simulink model "afe_rst_inv_psm_distributed_control_two_delays"  (R2026a)
settings: Solver=ode1be  StopTime=simlength  FixedStep=tc  MaxStep=Tc
values from neighbouring files (symbols this model uses):
  Amplitude_U = 1.16    [grid_fault_generator.m]
  Amplitude_V = Amplitude_U    (= 1.16)    [grid_fault_generator.m]
  Amplitude_W = Amplitude_U    (= 1.16)    [grid_fault_generator.m]
  end_time_LVRT = start_time_LVRT + error_length    [grid_fault_generator.m]
  Igrid_phase_normalization_factor = 270*sqrt(2)    [grid_emulator.m]
  omega_grid_emulator_nom = w_grid    (= 314.159265359)    [grid_emulator.m]
  omega_grid_nom = w_grid    (= 314.159265359)    [grid_emulator.m]
  t_ramp = 20e-3    (= 0.02)    [grid_fault_generator.m]
  ugrid_factor = 1    [grid_emulator.m]
  V_phase_normalization_factor = Vgrid_phase_normalization_factor    [grid_emulator.m]
  Vdc_bez = 1070    [grid_emulator.m]
  Vemu_ref_norm = Vemu_ref * sqrt(2) / V_phase_normalization_factor    [grid_emulator.m]
  vn_eta_pu = 0    [grid_emulator.m]
  vn_xi_pu = 0    [grid_emulator.m]
  vp_xi_pu = 1    [grid_emulator.m]
undefined symbols (not defined in the file or in its folder): Adrso, Aresd, Bresd, CFi, CFu, Cresd, Crso, CTRPIFF_CLIP_RELEASE, dead_time_INV, emf_fb_p, emf_fb_p_ccaller_1, emf_fb_p_ccaller_2, emf_p, emf_p_ccaller_1, emf_p_ccaller_2, fPWM_INV, g0_161Hz, g0_500Hz, g1_161Hz, g1_500Hz, i_grid_neg_eta_lim, i_grid_neg_eta_red_lim, i_grid_neg_xi_lim, i_grid_neg_xi_red_lim, i_grid_pos_eta_lim, i_grid_pos_eta_red_lim, ibez, id_lim, ieta_neg_ref_lim, ieta_pos_ref_lim, iq_lim, ixi_pos_ref_lim, Jm_norm, k_frt_ref, kg, ki_afe, ki_i, ki_id, ki_iq, ki_rc_neg_grid, ki_rc_pos_grid, ki_vs, ki_w, kp_afe, kp_i, kp_id, kp_iq, kp_rc_neg_grid, kp_rc_pos_grid, kp_vs, kp_w, kw, l1, l2, Lalpha_norm, Ld_norm, Ldrso, Lq_norm, Ls_norm, luenberger_l1 ... (+30)
libraries: fl_lib x146, nesl_utility x62, simulink x8, cstblocks_lti x7, sl_discontinuities x3, single_phase_transformer_lib x3, flexshaft_lib x1, permanent_magnet_synchronous_machine x1
(part 4 of 14)

== system afe_rst_inv_psm_distributed_control_two_delays/grid/instantaneus_power/moving_avarage1 ==
  In : Inport
  Gain1 : Gain  Gain=omega_grid_emulator_nom/2/pi  SaturateOnIntegerOverflow=on  OutDataTypeStr=Inherit: Same as input  ParamDataTypeStr=Inherit: Same as input
  Sum4 : Sum  SaturateOnIntegerOverflow=on
  Sum8 : Sum  Inputs=+-  InputSameDT=on  SaturateOnIntegerOverflow=on  OutDataTypeStr=Inherit: Same as first input
  Transport Delay : TransportDelay  DelayTime=2*pi/omega_grid_emulator_nom  BufferSize=2048*4  PadeOrder=2
  Unit Delay2 : UnitDelay  SampleTime=ts_afe
  kp2 : Gain  Gain=ts_afe  SaturateOnIntegerOverflow=on  OutDataTypeStr=Inherit: Same as input  ParamDataTypeStr=Inherit: Same as input
  Mean : Outport  VectorParamsAs1DForOutWhenUnconnected=off
  wires:
  Gain1/1 -> Mean/1
  kp2/1 -> Sum4/1
  Unit Delay2/1 -> Sum4/2
  In/1 -> kp2/1
  Sum8/1 -> Gain1/1
  Sum4/1 -> Unit Delay2/1, Transport Delay/1, Sum8/1
  Transport Delay/1 -> Sum8/2

== system afe_rst_inv_psm_distributed_control_two_delays/grid/instantaneus_power/rms ==
  In1 : Inport
  Gain : Gain  Gain=n10-1
  Gain1 : Gain  Gain=1/n10
  Math Function : Math  Operator=magnitude^2  SignedPower=on
  Sqrt : Sqrt
  Sum : Sum  Inputs=|++
  Unit Delay : UnitDelay  SampleTime=ts_afe
  Out1 : Outport  VectorParamsAs1DForOutWhenUnconnected=off
  wires:
  In1/1 -> Math Function/1
  Sum/1 -> Gain1/1
  Gain1/1 -> Sqrt/1, Unit Delay/1
  Unit Delay/1 -> Gain/1
  Math Function/1 -> Sum/1
  Sqrt/1 -> Out1/1
  Gain/1 -> Sum/2

== system afe_rst_inv_psm_distributed_control_two_delays/grid/instantaneus_power/rms1 ==
  In1 : Inport
  Gain : Gain  Gain=n10-1
  Gain1 : Gain  Gain=1/n10
  Math Function : Math  Operator=magnitude^2  SignedPower=on
  Sqrt : Sqrt
  Sum : Sum  Inputs=|++
  Unit Delay : UnitDelay  SampleTime=ts_afe
  Out1 : Outport  VectorParamsAs1DForOutWhenUnconnected=off
  wires:
  Gain/1 -> Sum/2
  Sqrt/1 -> Out1/1
  Math Function/1 -> Sum/1
  Unit Delay/1 -> Gain/1
  Gain1/1 -> Unit Delay/1, Sqrt/1
  Sum/1 -> Gain1/1
  In1/1 -> Math Function/1

== system afe_rst_inv_psm_distributed_control_two_delays/grid/instantaneus_power/rms2 ==
  In1 : Inport
  Gain : Gain  Gain=n10-1
  Gain1 : Gain  Gain=1/n10
  Math Function : Math  Operator=magnitude^2  SignedPower=on
  Sqrt : Sqrt
  Sum : Sum  Inputs=|++
  Unit Delay : UnitDelay  SampleTime=ts_afe
  Out1 : Outport  VectorParamsAs1DForOutWhenUnconnected=off
  wires:
  In1/1 -> Math Function/1
  Sum/1 -> Gain1/1
  Gain1/1 -> Sqrt/1, Unit Delay/1
  Unit Delay/1 -> Gain/1
  Math Function/1 -> Sum/1
  Sqrt/1 -> Out1/1
  Gain/1 -> Sum/2

== system afe_rst_inv_psm_distributed_control_two_delays/grid/instantaneus_power/rms3 ==
  In1 : Inport
  Gain : Gain  Gain=n10-1
  Gain1 : Gain  Gain=1/n10
  Math Function : Math  Operator=magnitude^2  SignedPower=on
  Sqrt : Sqrt
  Sum : Sum  Inputs=|++
  Unit Delay : UnitDelay  SampleTime=ts_afe
  Out1 : Outport  VectorParamsAs1DForOutWhenUnconnected=off
  wires:
  Gain/1 -> Sum/2
  Sqrt/1 -> Out1/1
  Math Function/1 -> Sum/1
  Unit Delay/1 -> Gain/1
  Gain1/1 -> Unit Delay/1, Sqrt/1
  Sum/1 -> Gain1/1
  In1/1 -> Math Function/1

== system afe_rst_inv_psm_distributed_control_two_delays/grid/instantaneus_power/rms4 ==
  In1 : Inport
  Gain : Gain  Gain=n10-1
  Gain1 : Gain  Gain=1/n10
  Math Function : Math  Operator=magnitude^2  SignedPower=on
  Sqrt : Sqrt
  Sum : Sum  Inputs=|++
  Unit Delay : UnitDelay  SampleTime=ts_afe
  Out1 : Outport  VectorParamsAs1DForOutWhenUnconnected=off
  wires:
  In1/1 -> Math Function/1
  Sum/1 -> Gain1/1
  Gain1/1 -> Sqrt/1, Unit Delay/1
  Unit Delay/1 -> Gain/1
  Math Function/1 -> Sum/1
  Sqrt/1 -> Out1/1
  Gain/1 -> Sum/2

== system afe_rst_inv_psm_distributed_control_two_delays/grid/instantaneus_power/rms5 ==
  In1 : Inport
  Gain : Gain  Gain=n10-1
  Gain1 : Gain  Gain=1/n10
  Math Function : Math  Operator=magnitude^2  SignedPower=on
  Sqrt : Sqrt
  Sum : Sum  Inputs=|++
  Unit Delay : UnitDelay  SampleTime=ts_afe
  Out1 : Outport  VectorParamsAs1DForOutWhenUnconnected=off
  wires:
  Gain/1 -> Sum/2
  Sqrt/1 -> Out1/1
  Math Function/1 -> Sum/1
  Unit Delay/1 -> Gain/1
  Gain1/1 -> Unit Delay/1, Sqrt/1
  Sum/1 -> Gain1/1
  In1/1 -> Math Function/1

== system afe_rst_inv_psm_distributed_control_two_delays/grid/sequences accordind to VDE411/moving_avarage ==
  In : Inport
  Gain1 : Gain  Gain=omega_grid_emulator_nom/2/pi  SaturateOnIntegerOverflow=on  OutDataTypeStr=Inherit: Same as input  ParamDataTypeStr=Inherit: Same as input
  Sum4 : Sum  SaturateOnIntegerOverflow=on
  Sum8 : Sum  Inputs=+-  InputSameDT=on  SaturateOnIntegerOverflow=on  OutDataTypeStr=Inherit: Same as first input
  Transport Delay : TransportDelay  DelayTime=2*pi/omega_grid_emulator_nom  BufferSize=2048*4  PadeOrder=2
  Unit Delay2 : UnitDelay  SampleTime=ts_afe
  kp2 : Gain  Gain=ts_afe  SaturateOnIntegerOverflow=on  OutDataTypeStr=Inherit: Same as input  ParamDataTypeStr=Inherit: Same as input
  Mean : Outport  VectorParamsAs1DForOutWhenUnconnected=off
  wires:
  Transport Delay/1 -> Sum8/2
  Sum4/1 -> Sum8/1, Transport Delay/1, Unit Delay2/1
  Sum8/1 -> Gain1/1
  In/1 -> kp2/1
  Unit Delay2/1 -> Sum4/2
  kp2/1 -> Sum4/1
  Gain1/1 -> Mean/1

== system afe_rst_inv_psm_distributed_control_two_delays/grid/sequences accordind to VDE411/moving_avarage1 ==
  In : Inport
  Gain1 : Gain  Gain=omega_grid_emulator_nom/2/pi  SaturateOnIntegerOverflow=on  OutDataTypeStr=Inherit: Same as input  ParamDataTypeStr=Inherit: Same as input
  Sum4 : Sum  SaturateOnIntegerOverflow=on
  Sum8 : Sum  Inputs=+-  InputSameDT=on  SaturateOnIntegerOverflow=on  OutDataTypeStr=Inherit: Same as first input
  Transport Delay : TransportDelay  DelayTime=2*pi/omega_grid_emulator_nom  BufferSize=2048*4  PadeOrder=2
  Unit Delay2 : UnitDelay  SampleTime=ts_afe
  kp2 : Gain  Gain=ts_afe  SaturateOnIntegerOverflow=on  OutDataTypeStr=Inherit: Same as input  ParamDataTypeStr=Inherit: Same as input
  Mean : Outport  VectorParamsAs1DForOutWhenUnconnected=off
  wires:
  Gain1/1 -> Mean/1
  kp2/1 -> Sum4/1
  Unit Delay2/1 -> Sum4/2
  In/1 -> kp2/1
  Sum8/1 -> Gain1/1
  Sum4/1 -> Unit Delay2/1, Transport Delay/1, Sum8/1
  Transport Delay/1 -> Sum8/2

== system afe_rst_inv_psm_distributed_control_two_delays/grid/sequences accordind to VDE411/moving_avarage10 ==
  In : Inport
  Gain1 : Gain  Gain=omega_grid_emulator_nom/2/pi  SaturateOnIntegerOverflow=on  OutDataTypeStr=Inherit: Same as input  ParamDataTypeStr=Inherit: Same as input
  Sum4 : Sum  SaturateOnIntegerOverflow=on
  Sum8 : Sum  Inputs=+-  InputSameDT=on  SaturateOnIntegerOverflow=on  OutDataTypeStr=Inherit: Same as first input
  Transport Delay : TransportDelay  DelayTime=2*pi/omega_grid_emulator_nom  BufferSize=2048*4  PadeOrder=2
  Unit Delay2 : UnitDelay  SampleTime=ts_afe
  kp2 : Gain  Gain=ts_afe  SaturateOnIntegerOverflow=on  OutDataTypeStr=Inherit: Same as input  ParamDataTypeStr=Inherit: Same as input
  Mean : Outport  VectorParamsAs1DForOutWhenUnconnected=off
  wires:
  Transport Delay/1 -> Sum8/2
  Sum4/1 -> Sum8/1, Transport Delay/1, Unit Delay2/1
  Sum8/1 -> Gain1/1
  In/1 -> kp2/1
  Unit Delay2/1 -> Sum4/2
  kp2/1 -> Sum4/1
  Gain1/1 -> Mean/1

== system afe_rst_inv_psm_distributed_control_two_delays/grid/sequences accordind to VDE411/moving_avarage11 ==
  In : Inport
  Gain1 : Gain  Gain=omega_grid_emulator_nom/2/pi  SaturateOnIntegerOverflow=on  OutDataTypeStr=Inherit: Same as input  ParamDataTypeStr=Inherit: Same as input
  Sum4 : Sum  SaturateOnIntegerOverflow=on
  Sum8 : Sum  Inputs=+-  InputSameDT=on  SaturateOnIntegerOverflow=on  OutDataTypeStr=Inherit: Same as first input
  Transport Delay : TransportDelay  DelayTime=2*pi/omega_grid_emulator_nom  BufferSize=2048*4  PadeOrder=2
  Unit Delay2 : UnitDelay  SampleTime=ts_afe
  kp2 : Gain  Gain=ts_afe  SaturateOnIntegerOverflow=on  OutDataTypeStr=Inherit: Same as input  ParamDataTypeStr=Inherit: Same as input
  Mean : Outport  VectorParamsAs1DForOutWhenUnconnected=off
  wires:
  Gain1/1 -> Mean/1
  kp2/1 -> Sum4/1
  Unit Delay2/1 -> Sum4/2
  In/1 -> kp2/1
  Sum8/1 -> Gain1/1
  Sum4/1 -> Unit Delay2/1, Transport Delay/1, Sum8/1
  Transport Delay/1 -> Sum8/2

== system afe_rst_inv_psm_distributed_control_two_delays/grid/sequences accordind to VDE411/moving_avarage2 ==
  In : Inport
  Gain1 : Gain  Gain=omega_grid_emulator_nom/2/pi  SaturateOnIntegerOverflow=on  OutDataTypeStr=Inherit: Same as input  ParamDataTypeStr=Inherit: Same as input
  Sum4 : Sum  SaturateOnIntegerOverflow=on
  Sum8 : Sum  Inputs=+-  InputSameDT=on  SaturateOnIntegerOverflow=on  OutDataTypeStr=Inherit: Same as first input
  Transport Delay : TransportDelay  DelayTime=2*pi/omega_grid_emulator_nom  BufferSize=2048*4  PadeOrder=2
  Unit Delay2 : UnitDelay  SampleTime=ts_afe
  kp2 : Gain  Gain=ts_afe  SaturateOnIntegerOverflow=on  OutDataTypeStr=Inherit: Same as input  ParamDataTypeStr=Inherit: Same as input
  Mean : Outport  VectorParamsAs1DForOutWhenUnconnected=off
  wires:
  Transport Delay/1 -> Sum8/2
  Sum4/1 -> Sum8/1, Transport Delay/1, Unit Delay2/1
  Sum8/1 -> Gain1/1
  In/1 -> kp2/1
  Unit Delay2/1 -> Sum4/2
  kp2/1 -> Sum4/1
  Gain1/1 -> Mean/1

== system afe_rst_inv_psm_distributed_control_two_delays/grid/sequences accordind to VDE411/moving_avarage3 ==
  In : Inport
  Gain1 : Gain  Gain=omega_grid_emulator_nom/2/pi  SaturateOnIntegerOverflow=on  OutDataTypeStr=Inherit: Same as input  ParamDataTypeStr=Inherit: Same as input
  Sum4 : Sum  SaturateOnIntegerOverflow=on
  Sum8 : Sum  Inputs=+-  InputSameDT=on  SaturateOnIntegerOverflow=on  OutDataTypeStr=Inherit: Same as first input
  Transport Delay : TransportDelay  DelayTime=2*pi/omega_grid_emulator_nom  BufferSize=2048*4  PadeOrder=2
  Unit Delay2 : UnitDelay  SampleTime=ts_afe
  kp2 : Gain  Gain=ts_afe  SaturateOnIntegerOverflow=on  OutDataTypeStr=Inherit: Same as input  ParamDataTypeStr=Inherit: Same as input
  Mean : Outport  VectorParamsAs1DForOutWhenUnconnected=off
  wires:
  Gain1/1 -> Mean/1
  kp2/1 -> Sum4/1
  Unit Delay2/1 -> Sum4/2
  In/1 -> kp2/1
  Sum8/1 -> Gain1/1
  Sum4/1 -> Unit Delay2/1, Transport Delay/1, Sum8/1
  Transport Delay/1 -> Sum8/2

== system afe_rst_inv_psm_distributed_control_two_delays/grid/sequences accordind to VDE411/moving_avarage4 ==
  In : Inport
  Gain1 : Gain  Gain=omega_grid_emulator_nom/2/pi  SaturateOnIntegerOverflow=on  OutDataTypeStr=Inherit: Same as input  ParamDataTypeStr=Inherit: Same as input
  Sum4 : Sum  SaturateOnIntegerOverflow=on
  Sum8 : Sum  Inputs=+-  InputSameDT=on  SaturateOnIntegerOverflow=on  OutDataTypeStr=Inherit: Same as first input
  Transport Delay : TransportDelay  DelayTime=2*pi/omega_grid_emulator_nom  BufferSize=2048*4  PadeOrder=2
  Unit Delay2 : UnitDelay  SampleTime=ts_afe
  kp2 : Gain  Gain=ts_afe  SaturateOnIntegerOverflow=on  OutDataTypeStr=Inherit: Same as input  ParamDataTypeStr=Inherit: Same as input
  Mean : Outport  VectorParamsAs1DForOutWhenUnconnected=off
  wires:
  Transport Delay/1 -> Sum8/2
  Sum4/1 -> Sum8/1, Transport Delay/1, Unit Delay2/1
  Sum8/1 -> Gain1/1
  In/1 -> kp2/1
  Unit Delay2/1 -> Sum4/2
  kp2/1 -> Sum4/1
  Gain1/1 -> Mean/1

== system afe_rst_inv_psm_distributed_control_two_delays/grid/sequences accordind to VDE411/moving_avarage5 ==
  In : Inport
  Gain1 : Gain  Gain=omega_grid_emulator_nom/2/pi  SaturateOnIntegerOverflow=on  OutDataTypeStr=Inherit: Same as input  ParamDataTypeStr=Inherit: Same as input
  Sum4 : Sum  SaturateOnIntegerOverflow=on
  Sum8 : Sum  Inputs=+-  InputSameDT=on  SaturateOnIntegerOverflow=on  OutDataTypeStr=Inherit: Same as first input
  Transport Delay : TransportDelay  DelayTime=2*pi/omega_grid_emulator_nom  BufferSize=2048*4  PadeOrder=2
  Unit Delay2 : UnitDelay  SampleTime=ts_afe
  kp2 : Gain  Gain=ts_afe  SaturateOnIntegerOverflow=on  OutDataTypeStr=Inherit: Same as input  ParamDataTypeStr=Inherit: Same as input
  Mean : Outport  VectorParamsAs1DForOutWhenUnconnected=off
  wires:
  Gain1/1 -> Mean/1
  kp2/1 -> Sum4/1
  Unit Delay2/1 -> Sum4/2
  In/1 -> kp2/1
  Sum8/1 -> Gain1/1
  Sum4/1 -> Unit Delay2/1, Transport Delay/1, Sum8/1
  Transport Delay/1 -> Sum8/2

== system afe_rst_inv_psm_distributed_control_two_delays/grid/sequences accordind to VDE411/moving_avarage6 ==
  In : Inport
  Gain1 : Gain  Gain=omega_grid_emulator_nom/2/pi  SaturateOnIntegerOverflow=on  OutDataTypeStr=Inherit: Same as input  ParamDataTypeStr=Inherit: Same as input
  Sum4 : Sum  SaturateOnIntegerOverflow=on
  Sum8 : Sum  Inputs=+-  InputSameDT=on  SaturateOnIntegerOverflow=on  OutDataTypeStr=Inherit: Same as first input
  Transport Delay : TransportDelay  DelayTime=2*pi/omega_grid_emulator_nom  BufferSize=2048*4  PadeOrder=2
  Unit Delay2 : UnitDelay  SampleTime=ts_afe
  kp2 : Gain  Gain=ts_afe  SaturateOnIntegerOverflow=on  OutDataTypeStr=Inherit: Same as input  ParamDataTypeStr=Inherit: Same as input
  Mean : Outport  VectorParamsAs1DForOutWhenUnconnected=off
  wires:
  Transport Delay/1 -> Sum8/2
  Sum4/1 -> Sum8/1, Transport Delay/1, Unit Delay2/1
  Sum8/1 -> Gain1/1
  In/1 -> kp2/1
  Unit Delay2/1 -> Sum4/2
  kp2/1 -> Sum4/1
  Gain1/1 -> Mean/1

== system afe_rst_inv_psm_distributed_control_two_delays/grid/sequences accordind to VDE411/moving_avarage7 ==
  In : Inport
  Gain1 : Gain  Gain=omega_grid_emulator_nom/2/pi  SaturateOnIntegerOverflow=on  OutDataTypeStr=Inherit: Same as input  ParamDataTypeStr=Inherit: Same as input
  Sum4 : Sum  SaturateOnIntegerOverflow=on
  Sum8 : Sum  Inputs=+-  InputSameDT=on  SaturateOnIntegerOverflow=on  OutDataTypeStr=Inherit: Same as first input
  Transport Delay : TransportDelay  DelayTime=2*pi/omega_grid_emulator_nom  BufferSize=2048*4  PadeOrder=2
  Unit Delay2 : UnitDelay  SampleTime=ts_afe
  kp2 : Gain  Gain=ts_afe  SaturateOnIntegerOverflow=on  OutDataTypeStr=Inherit: Same as input  ParamDataTypeStr=Inherit: Same as input
  Mean : Outport  VectorParamsAs1DForOutWhenUnconnected=off
  wires:
  Gain1/1 -> Mean/1
  kp2/1 -> Sum4/1
  Unit Delay2/1 -> Sum4/2
  In/1 -> kp2/1
  Sum8/1 -> Gain1/1
  Sum4/1 -> Unit Delay2/1, Transport Delay/1, Sum8/1
  Transport Delay/1 -> Sum8/2

== system afe_rst_inv_psm_distributed_control_two_delays/grid/sequences accordind to VDE411/moving_avarage8 ==
  In : Inport
  Gain1 : Gain  Gain=omega_grid_emulator_nom/2/pi  SaturateOnIntegerOverflow=on  OutDataTypeStr=Inherit: Same as input  ParamDataTypeStr=Inherit: Same as input
  Sum4 : Sum  SaturateOnIntegerOverflow=on
  Sum8 : Sum  Inputs=+-  InputSameDT=on  SaturateOnIntegerOverflow=on  OutDataTypeStr=Inherit: Same as first input
  Transport Delay : TransportDelay  DelayTime=2*pi/omega_grid_emulator_nom  BufferSize=2048*4  PadeOrder=2
  Unit Delay2 : UnitDelay  SampleTime=ts_afe
  kp2 : Gain  Gain=ts_afe  SaturateOnIntegerOverflow=on  OutDataTypeStr=Inherit: Same as input  ParamDataTypeStr=Inherit: Same as input
  Mean : Outport  VectorParamsAs1DForOutWhenUnconnected=off
  wires:
  Transport Delay/1 -> Sum8/2
  Sum4/1 -> Sum8/1, Transport Delay/1, Unit Delay2/1
  Sum8/1 -> Gain1/1
  In/1 -> kp2/1
  Unit Delay2/1 -> Sum4/2
  kp2/1 -> Sum4/1
  Gain1/1 -> Mean/1

== system afe_rst_inv_psm_distributed_control_two_delays/grid/sequences accordind to VDE411/moving_avarage9 ==
  In : Inport
  Gain1 : Gain  Gain=omega_grid_emulator_nom/2/pi  SaturateOnIntegerOverflow=on  OutDataTypeStr=Inherit: Same as input  ParamDataTypeStr=Inherit: Same as input
  Sum4 : Sum  SaturateOnIntegerOverflow=on
  Sum8 : Sum  Inputs=+-  InputSameDT=on  SaturateOnIntegerOverflow=on  OutDataTypeStr=Inherit: Same as first input
  Transport Delay : TransportDelay  DelayTime=2*pi/omega_grid_emulator_nom  BufferSize=2048*4  PadeOrder=2
  Unit Delay2 : UnitDelay  SampleTime=ts_afe
  kp2 : Gain  Gain=ts_afe  SaturateOnIntegerOverflow=on  OutDataTypeStr=Inherit: Same as input  ParamDataTypeStr=Inherit: Same as input
  Mean : Outport  VectorParamsAs1DForOutWhenUnconnected=off
  wires:
  Gain1/1 -> Mean/1
  kp2/1 -> Sum4/1
  Unit Delay2/1 -> Sum4/2
  In/1 -> kp2/1
  Sum8/1 -> Gain1/1
  Sum4/1 -> Unit Delay2/1, Transport Delay/1, Sum8/1
  Transport Delay/1 -> Sum8/2

== system afe_rst_inv_psm_distributed_control_two_delays/mainboard_afe/current_sequence_avg/Moving Average Filter5 ==
  In2 : Inport
  In3 : Inport  Port=2
  Bus Selector : BusSelector  OutputSignals=ts,sshort,slong,pinput,cbpointer,cbsample,mavg_output
  C Caller : CCaller  FunctionName=mavgflt_process_simulink  PortSpecificationStruct="%)30     .    B H   8    (     @         %    \"     8    !     0         %  0 \"0    $    _    07)G3F%M90  4&]R=$YA;64 4V-O<&4     26YD97@     5'EP90      4VEZ90      27-';&]B86P   X    P    !@    @    $          4    (     0    ,    !         !   P!O=70 #@   #     &    \"     0         !0    @    !     P    $         $  # &]U=  .    .     8    (    !          %    \"     $    &     0         0   ...(+3251 chars)"  SampleTime=ts_afe
  Compare To Zero : simulink/Logic and Bit Operations/Compare To Zero  relop=>  OutDataTypeStr=boolean
  Constant : Constant  Value=5
  Constant5 : Constant  Value=ts_afe
  Data Type Conversion : DataTypeConversion  OutDataTypeStr=single  SaturateOnIntegerOverflow=off  RndMeth=Floor
  Data Type Conversion1 : DataTypeConversion  OutDataTypeStr=single  SaturateOnIntegerOverflow=off  RndMeth=Floor
  Data Type Conversion2 : DataTypeConversion  OutDataTypeStr=single  SaturateOnIntegerOverflow=off  RndMeth=Floor
  Data Type Conversion3 : DataTypeConversion  OutDataTypeStr=double  SaturateOnIntegerOverflow=off  RndMeth=Floor
  Data Type Conversion4 : DataTypeConversion  OutDataTypeStr=uint8  SaturateOnIntegerOverflow=off  RndMeth=Floor
  Data Type Conversion5 : DataTypeConversion  OutDataTypeStr=uint8  SaturateOnIntegerOverflow=off  RndMeth=Floor
  Enabled Subsystem : Subsystem  TreatAsAtomicUnit=on
  Reset Trigger : Subsystem
  Terminator{,1..5} (6 alike) : Terminator
  Zero-Order Hold1 : ZeroOrderHold  SampleTime=ts_afe
  Zero-Order Hold2 : ZeroOrderHold  SampleTime=ts_afe
  xi : Outport
  wires:
  Bus Selector/5 -> Terminator2/1  "<cbpointer>"
  Bus Selector/4 -> Terminator1/1  "<pinput>"
  Data Type Conversion3/1 -> xi/1  "output"
  Zero-Order Hold2/1 -> Data Type Conversion/1  "d1"
  Enabled Subsystem/1(Out1) -> Data Type Conversion1/1
  Compare To Zero/1 -> Enabled Subsystem/Enable
  In3/1 -> Enabled Subsystem/1(In1), Compare To Zero/1  "omega_grid"
  Constant5/1 -> Zero-Order Hold1/1
  Zero-Order Hold1/1 -> Data Type Conversion2/1  "d1"
  Bus Selector/3 -> Terminator4/1  "<slong>"
  Bus Selector/2 -> Terminator3/1  "<sshort>"
  Bus Selector/1 -> Terminator/1  "<ts>"
  C Caller/1 -> Bus Selector/1  "out"
  In2/1 -> Zero-Order Hold2/1  "input"
  Data Type Conversion4/1 -> C Caller/5
  Data Type Conversion/1 -> C Caller/1  "input"
  Data Type Conversion5/1 -> C Caller/4
  Data Type Conversion2/1 -> C Caller/3
  Data Type Conversion1/1 -> C Caller/2
  Reset Trigger/1(Out1) -> Data Type Conversion5/1
  Constant/1 -> Data Type Conversion4/1
  Bus Selector/6 -> Terminator5/1  "<cbsample>"
  Bus Selector/7 -> Data Type Conversion3/1  "<mavg_output>"

== system afe_rst_inv_psm_distributed_control_two_delays/mainboard_afe/current_sequence_avg/Moving Average Filter6 ==
  In2 : Inport
  In3 : Inport  Port=2
  Bus Selector : BusSelector  OutputSignals=ts,sshort,slong,pinput,cbpointer,cbsample,mavg_output
  C Caller : CCaller  FunctionName=mavgflt_process_simulink  PortSpecificationStruct="%)30     .    B H   8    (     @         %    \"     8    !     0         %  0 \"0    $    _    07)G3F%M90  4&]R=$YA;64 4V-O<&4     26YD97@     5'EP90      4VEZ90      27-';&]B86P   X    P    !@    @    $          4    (     0    ,    !         !   P!O=70 #@   #     &    \"     0         !0    @    !     P    $         $  # &]U=  .    .     8    (    !          %    \"     $    &     0         0   ...(+3251 chars)"  SampleTime=ts_afe
  Compare To Zero : simulink/Logic and Bit Operations/Compare To Zero  relop=>  OutDataTypeStr=boolean
  Constant : Constant  Value=6
  Constant5 : Constant  Value=ts_afe
  Data Type Conversion : DataTypeConversion  OutDataTypeStr=single  SaturateOnIntegerOverflow=off  RndMeth=Floor
  Data Type Conversion1 : DataTypeConversion  OutDataTypeStr=single  SaturateOnIntegerOverflow=off  RndMeth=Floor
  Data Type Conversion2 : DataTypeConversion  OutDataTypeStr=single  SaturateOnIntegerOverflow=off  RndMeth=Floor
  Data Type Conversion3 : DataTypeConversion  OutDataTypeStr=double  SaturateOnIntegerOverflow=off  RndMeth=Floor
  Data Type Conversion4 : DataTypeConversion  OutDataTypeStr=uint8  SaturateOnIntegerOverflow=off  RndMeth=Floor
  Data Type Conversion5 : DataTypeConversion  OutDataTypeStr=uint8  SaturateOnIntegerOverflow=off  RndMeth=Floor
  Enabled Subsystem : Subsystem  TreatAsAtomicUnit=on
  Reset Trigger : Subsystem
  Terminator{,1..5} (6 alike) : Terminator
  Zero-Order Hold1 : ZeroOrderHold  SampleTime=ts_afe
  Zero-Order Hold2 : ZeroOrderHold  SampleTime=ts_afe
  xi : Outport
  wires:
  Bus Selector/7 -> Data Type Conversion3/1  "<mavg_output>"
  Bus Selector/6 -> Terminator5/1  "<cbsample>"
  Constant/1 -> Data Type Conversion4/1
  Reset Trigger/1(Out1) -> Data Type Conversion5/1
  Data Type Conversion1/1 -> C Caller/2
  Data Type Conversion2/1 -> C Caller/3
  Data Type Conversion5/1 -> C Caller/4
  Data Type Conversion/1 -> C Caller/1  "input"
  Data Type Conversion4/1 -> C Caller/5
  In2/1 -> Zero-Order Hold2/1  "input"
  C Caller/1 -> Bus Selector/1  "out"
  Bus Selector/1 -> Terminator/1  "<ts>"
  Bus Selector/2 -> Terminator3/1  "<sshort>"
  Bus Selector/3 -> Terminator4/1  "<slong>"
  Zero-Order Hold1/1 -> Data Type Conversion2/1  "d1"
  Constant5/1 -> Zero-Order Hold1/1
  In3/1 -> Compare To Zero/1, Enabled Subsystem/1(In1)  "omega_grid"
  Compare To Zero/1 -> Enabled Subsystem/Enable
  Enabled Subsystem/1(Out1) -> Data Type Conversion1/1
  Zero-Order Hold2/1 -> Data Type Conversion/1  "d1"
  Data Type Conversion3/1 -> xi/1  "output"
  Bus Selector/4 -> Terminator1/1  "<pinput>"
  Bus Selector/5 -> Terminator2/1  "<cbpointer>"

== system afe_rst_inv_psm_distributed_control_two_delays/mainboard_afe/current_sequence_avg/Moving Average Filter7 ==
  In2 : Inport
  In3 : Inport  Port=2
  Bus Selector : BusSelector  OutputSignals=ts,sshort,slong,pinput,cbpointer,cbsample,mavg_output
  C Caller : CCaller  FunctionName=mavgflt_process_simulink  PortSpecificationStruct="%)30     .    B H   8    (     @         %    \"     8    !     0         %  0 \"0    $    _    07)G3F%M90  4&]R=$YA;64 4V-O<&4     26YD97@     5'EP90      4VEZ90      27-';&]B86P   X    P    !@    @    $          4    (     0    ,    !         !   P!O=70 #@   #     &    \"     0         !0    @    !     P    $         $  # &]U=  .    .     8    (    !          %    \"     $    &     0         0   ...(+3251 chars)"  SampleTime=ts_afe
  Compare To Zero : simulink/Logic and Bit Operations/Compare To Zero  relop=>  OutDataTypeStr=boolean
  Constant : Constant  Value=7
  Constant5 : Constant  Value=ts_afe
  Data Type Conversion : DataTypeConversion  OutDataTypeStr=single  SaturateOnIntegerOverflow=off  RndMeth=Floor
  Data Type Conversion1 : DataTypeConversion  OutDataTypeStr=single  SaturateOnIntegerOverflow=off  RndMeth=Floor
  Data Type Conversion2 : DataTypeConversion  OutDataTypeStr=single  SaturateOnIntegerOverflow=off  RndMeth=Floor
  Data Type Conversion3 : DataTypeConversion  OutDataTypeStr=double  SaturateOnIntegerOverflow=off  RndMeth=Floor
  Data Type Conversion4 : DataTypeConversion  OutDataTypeStr=uint8  SaturateOnIntegerOverflow=off  RndMeth=Floor
  Data Type Conversion5 : DataTypeConversion  OutDataTypeStr=uint8  SaturateOnIntegerOverflow=off  RndMeth=Floor
  Enabled Subsystem : Subsystem  TreatAsAtomicUnit=on
  Reset Trigger : Subsystem
  Terminator{,1..5} (6 alike) : Terminator
  Zero-Order Hold1 : ZeroOrderHold  SampleTime=ts_afe
  Zero-Order Hold2 : ZeroOrderHold  SampleTime=ts_afe
  xi : Outport
  wires:
  Bus Selector/5 -> Terminator2/1  "<cbpointer>"
  Bus Selector/4 -> Terminator1/1  "<pinput>"
  Data Type Conversion3/1 -> xi/1  "output"
  Zero-Order Hold2/1 -> Data Type Conversion/1  "d1"
  Enabled Subsystem/1(Out1) -> Data Type Conversion1/1
  Compare To Zero/1 -> Enabled Subsystem/Enable
  In3/1 -> Enabled Subsystem/1(In1), Compare To Zero/1  "omega_grid"
  Constant5/1 -> Zero-Order Hold1/1
  Zero-Order Hold1/1 -> Data Type Conversion2/1  "d1"
  Bus Selector/3 -> Terminator4/1  "<slong>"
  Bus Selector/2 -> Terminator3/1  "<sshort>"
  Bus Selector/1 -> Terminator/1  "<ts>"
  C Caller/1 -> Bus Selector/1  "out"
  In2/1 -> Zero-Order Hold2/1  "input"
  Data Type Conversion4/1 -> C Caller/5
  Data Type Conversion/1 -> C Caller/1  "input"
  Data Type Conversion5/1 -> C Caller/4
  Data Type Conversion2/1 -> C Caller/3
  Data Type Conversion1/1 -> C Caller/2
  Reset Trigger/1(Out1) -> Data Type Conversion5/1
  Constant/1 -> Data Type Conversion4/1
  Bus Selector/6 -> Terminator5/1  "<cbsample>"
  Bus Selector/7 -> Data Type Conversion3/1  "<mavg_output>"

== system afe_rst_inv_psm_distributed_control_two_delays/mainboard_afe/current_sequence_avg/Moving Average Filter8 ==
  In2 : Inport
  In3 : Inport  Port=2
  Bus Selector : BusSelector  OutputSignals=ts,sshort,slong,pinput,cbpointer,cbsample,mavg_output
  C Caller : CCaller  FunctionName=mavgflt_process_simulink  PortSpecificationStruct="%)30     .    B H   8    (     @         %    \"     8    !     0         %  0 \"0    $    _    07)G3F%M90  4&]R=$YA;64 4V-O<&4     26YD97@     5'EP90      4VEZ90      27-';&]B86P   X    P    !@    @    $          4    (     0    ,    !         !   P!O=70 #@   #     &    \"     0         !0    @    !     P    $         $  # &]U=  .    .     8    (    !          %    \"     $    &     0         0   ...(+3251 chars)"  SampleTime=ts_afe
  Compare To Zero : simulink/Logic and Bit Operations/Compare To Zero  relop=>  OutDataTypeStr=boolean
  Constant : Constant  Value=8
  Constant5 : Constant  Value=ts_afe
  Data Type Conversion : DataTypeConversion  OutDataTypeStr=single  SaturateOnIntegerOverflow=off  RndMeth=Floor
  Data Type Conversion1 : DataTypeConversion  OutDataTypeStr=single  SaturateOnIntegerOverflow=off  RndMeth=Floor
  Data Type Conversion2 : DataTypeConversion  OutDataTypeStr=single  SaturateOnIntegerOverflow=off  RndMeth=Floor
  Data Type Conversion3 : DataTypeConversion  OutDataTypeStr=double  SaturateOnIntegerOverflow=off  RndMeth=Floor
  Data Type Conversion4 : DataTypeConversion  OutDataTypeStr=uint8  SaturateOnIntegerOverflow=off  RndMeth=Floor
  Data Type Conversion5 : DataTypeConversion  OutDataTypeStr=uint8  SaturateOnIntegerOverflow=off  RndMeth=Floor
  Enabled Subsystem : Subsystem  TreatAsAtomicUnit=on
  Reset Trigger : Subsystem
  Terminator{,1..5} (6 alike) : Terminator
  Zero-Order Hold1 : ZeroOrderHold  SampleTime=ts_afe
  Zero-Order Hold2 : ZeroOrderHold  SampleTime=ts_afe
  xi : Outport
  wires:
  Bus Selector/7 -> Data Type Conversion3/1  "<mavg_output>"
  Bus Selector/6 -> Terminator5/1  "<cbsample>"
  Constant/1 -> Data Type Conversion4/1
  Reset Trigger/1(Out1) -> Data Type Conversion5/1
  Data Type Conversion1/1 -> C Caller/2
  Data Type Conversion2/1 -> C Caller/3
  Data Type Conversion5/1 -> C Caller/4
  Data Type Conversion/1 -> C Caller/1  "input"
  Data Type Conversion4/1 -> C Caller/5
  In2/1 -> Zero-Order Hold2/1  "input"
  C Caller/1 -> Bus Selector/1  "out"
  Bus Selector/1 -> Terminator/1  "<ts>"
  Bus Selector/2 -> Terminator3/1  "<sshort>"
  Bus Selector/3 -> Terminator4/1  "<slong>"
  Zero-Order Hold1/1 -> Data Type Conversion2/1  "d1"
  Constant5/1 -> Zero-Order Hold1/1
  In3/1 -> Compare To Zero/1, Enabled Subsystem/1(In1)  "omega_grid"
  Compare To Zero/1 -> Enabled Subsystem/Enable
  Enabled Subsystem/1(Out1) -> Data Type Conversion1/1
  Zero-Order Hold2/1 -> Data Type Conversion/1  "d1"
  Data Type Conversion3/1 -> xi/1  "output"
  Bus Selector/4 -> Terminator1/1  "<pinput>"
  Bus Selector/5 -> Terminator2/1  "<cbpointer>"

== system afe_rst_inv_psm_distributed_control_two_delays/mainboard_afe/dq_pll/pll_stageA ==
  gamma_grid : Inport
  Math Function : Math  Operator=magnitude^2  SignedPower=on
  Math Function1 : Math  Operator=magnitude^2  SignedPower=on
  Reciprocal Sqrt : Sqrt  Operator=rSqrt
  Saturation : Saturate  UpperLimit=inf  LowerLimit=0.02
  Sum : Sum  Inputs=|++
  abc_to_alphabeta : Subsystem
  sequences : Subsystem
  u_grid_pos_xi : Outport  VectorParamsAs1DForOutWhenUnconnected=off
  u_grid_pos_eta : Outport  Port=2  VectorParamsAs1DForOutWhenUnconnected=off
  tag scope: Vgrid_unorm=global
  wires:
  abc_to_alphabeta/1(ug_alpha) -> Math Function/1, sequences/1(u_grid_alpha)
  abc_to_alphabeta/2(ug_beta) -> Math Function1/1, sequences/2(u_grid_beta)
  Math Function/1 -> Sum/1
  Math Function1/1 -> Sum/2
  Sum/1 -> Saturation/1
  Reciprocal Sqrt/1 -> [Vgrid_unorm]
  Saturation/1 -> Reciprocal Sqrt/1
  gamma_grid/1 -> sequences/3(gamma_grid)
  sequences/1(u_grid_pos_xi) -> u_grid_pos_xi/1
  sequences/2(u_grid_pos_eta) -> u_grid_pos_eta/1
  [uga_pu_dba_fb_mbafe] -> abc_to_alphabeta/1(ug_a)
  [ugb_pu_dbb_fb_mbafe] -> abc_to_alphabeta/2(ug_b)
  [ugc_pu_dbc_fb_mbafe] -> abc_to_alphabeta/3(ug_c)

== system afe_rst_inv_psm_distributed_control_two_delays/mainboard_afe/dq_pll/pll_stageB ==
  u_grid_pos_xi : Inport
  u_grid_pos_eta : Inport  Port=2
  -2<x<2 : Saturate  UpperLimit=2  LowerLimit=-2
  Constant4 : Constant  Value=omega_grid_nom
  Product1 : Product  RndMeth=Zero
  Product2 : Product  RndMeth=Zero
  Sum3 : Sum  SaturateOnIntegerOverflow=on
  Sum4 : Sum  SaturateOnIntegerOverflow=on
  Sum5 : Sum  Inputs=++|
  To Workspace1 : ToWorkspace  VariableName=omega_grid_pll_sim  SampleTime=ts_afe
      settings: MaxDataPoints=Ns_afe
  To Workspace5 : ToWorkspace  VariableName=vgrid_xi_pll_pos_sim  SampleTime=ts_afe
      settings: MaxDataPoints=Ns_afe
  To Workspace6 : ToWorkspace  VariableName=vgrid_eta_pll_pos_sim  SampleTime=ts_afe
      settings: MaxDataPoints=Ns_afe
  To Workspace7 : ToWorkspace  VariableName=gamma_grid_pll_sim  SampleTime=ts_afe
      settings: MaxDataPoints=Ns_afe
  Unit Delay{1..5} (5 alike) : UnitDelay  SampleTime=ts_afe
  bounder1 : MATLAB Function  TreatAsAtomicUnit=on  SystemSampleTime=ts_afe
  double_integrator_observer : Subsystem
  kp : Gain  Gain=pll_i1*ts_afe  SaturateOnIntegerOverflow=on  OutDataTypeStr=Inherit: Same as input  ParamDataTypeStr=Inherit: Same as input
  kp1 : Gain  Gain=pll_p  SaturateOnIntegerOverflow=on  OutDataTypeStr=Inherit: Same as input  ParamDataTypeStr=Inherit: Same as input
  kp2 : Gain  Gain=ts_afe  SaturateOnIntegerOverflow=on  OutDataTypeStr=Inherit: Same as input  ParamDataTypeStr=Inherit: Same as input
  gamma_grid_pll : Outport  VectorParamsAs1DForOutWhenUnconnected=off
  tag scope: omega_grid_pll=global
  wires:
  Unit Delay4/1 -> Sum3/2, Sum5/2
  Sum3/1 -> -2<x<2/1
  Sum4/1 -> bounder1/1(u)
  Unit Delay1/1 -> Sum4/2
  -2<x<2/1 -> Unit Delay4/1  "i1"
  kp2/1 -> Sum4/1
  Constant4/1 -> Product2/2
  [Vgrid_unorm] -> Unit Delay3/1
  kp/1 -> Sum3/1
  Sum5/1 -> Product2/1
  bounder1/1(y) -> Unit Delay1/1, Unit Delay2/1
  u_grid_pos_xi/1 -> To Workspace5/1
  u_grid_pos_eta/1 -> Unit Delay5/1
  Product2/1 -> kp2/1
  Product1/1 -> kp/1, kp1/1  "V l"
  kp1/1 -> Sum5/1
  Unit Delay2/1 -> double_integrator_observer/1(theta), To Workspace7/1, gamma_grid_pll/1
  double_integrator_observer/1(omega_hat) -> To Workspace1/1, [omega_grid_pll]
  Unit Delay3/1 -> Product1/2
  Unit Delay5/1 -> To Workspace6/1, Product1/1

== system afe_rst_inv_psm_distributed_control_two_delays/mainboard_afe/grid_current_sampling_and_alpha_beta_transformation/iga_measure ==
  ig : Inport
  Bus Creator : BusCreator  Inputs=3
  Bus Selector : BusSelector  OutputSignals=iga,igb,igc
  Gain : Gain  Gain=1/Igrid_phase_normalization_factor
  Gain1 : Gain  Gain=1/Igrid_phase_normalization_factor
  Gain2 : Gain  Gain=1/Igrid_phase_normalization_factor
  Quantizer : Quantizer  QuantizationInterval=CurrentQuantization
  Quantizer1 : Quantizer  QuantizationInterval=CurrentQuantization
  Quantizer2 : Quantizer  QuantizationInterval=CurrentQuantization
  Unit Delay : UnitDelay  SampleTime=ts_afe
  Unit Delay1 : UnitDelay  SampleTime=ts_afe
  Unit Delay2 : UnitDelay  SampleTime=ts_afe
  Zero-Order Hold : ZeroOrderHold  SampleTime=ts_afe
  Zero-Order Hold1 : ZeroOrderHold  SampleTime=ts_afe
  Zero-Order Hold2 : ZeroOrderHold  SampleTime=ts_afe
  ig_pu : Outport
  wires:
  Quantizer/1 -> Zero-Order Hold/1
  Zero-Order Hold/1 -> Unit Delay/1
  Unit Delay/1 -> Gain/1
  ig/1 -> Bus Selector/1
  Bus Selector/1 -> Quantizer/1  "<iga>"
  Unit Delay1/1 -> Gain1/1
  Zero-Order Hold1/1 -> Unit Delay1/1
  Quantizer1/1 -> Zero-Order Hold1/1
  Bus Selector/2 -> Quantizer1/1  "<igb>"
  Quantizer2/1 -> Zero-Order Hold2/1
  Zero-Order Hold2/1 -> Unit Delay2/1
  Unit Delay2/1 -> Gain2/1
  Bus Selector/3 -> Quantizer2/1  "<igc>"
  Gain/1 -> Bus Creator/1
  Gain1/1 -> Bus Creator/2
  Gain2/1 -> Bus Creator/3
  Bus Creator/1 -> ig_pu/1

== system afe_rst_inv_psm_distributed_control_two_delays/mainboard_afe/sequences_current_control/negative_sequence_eta_current_control ==
  ff : Inport
  e : Inport  Port=2
  1/Ti : Gain  Gain=kp_rc_neg_grid  SaturateOnIntegerOverflow=on  OutDataTypeStr=Inherit: Same as input  ParamDataTypeStr=Inherit: Same as input
  1/Ti1 : Gain  SaturateOnIntegerOverflow=on  OutDataTypeStr=Inherit: Same as input  ParamDataTypeStr=Inherit: Same as input
  Saturation : Saturate  UpperLimit=ieta_neg_ref_lim  LowerLimit=-ieta_neg_ref_lim
  Sum : Sum  Inputs=|++
  Sum2 : Sum  Inputs=+++  SaturateOnIntegerOverflow=on
  Sum3 : Sum  Inputs=-+  SaturateOnIntegerOverflow=on
  Unit Delay1 : UnitDelay  SampleTime=ts_afe
  Unit Delay4 : UnitDelay  SampleTime=ts_afe
  kp : Gain  Gain=ki_rc_neg_grid*ts_afe  SaturateOnIntegerOverflow=on  OutDataTypeStr=Inherit: Same as input  ParamDataTypeStr=Inherit: Same as input
  u : Outport  VectorParamsAs1DForOutWhenUnconnected=off
  wires:
  Unit Delay4/1 -> Sum2/3
  Sum3/1 -> Unit Delay4/1
  kp/1 -> Sum2/2
  Sum2/1 -> Saturation/1
  1/Ti/1 -> Sum2/1, Sum3/1
  Saturation/1 -> Sum/1, Sum3/2
  Sum/1 -> Unit Delay1/1
  ff/1 -> 1/Ti1/1
  1/Ti1/1 -> Sum/2
  e/1 -> 1/Ti/1, kp/1  "e"
  Unit Delay1/1 -> u/1
